simulink model "USV_Battery_MPC_First_Evaluation"  (R2025b)
settings: Solver=ode45  StartTime=0.0  StopTime=1100  MaxStep=0.1  RelTol=1e-3
model workspace (MAT data in the model file):
  battery_aware_enable = 1
  controller_mode = 2
  initial_soc = 80
  params.usv.m = 120
  params.usv.Cd = 25
  params.usv.T_max = 200
  params.usv.T_min = 0
  params.usv.u_max = 3.5
  params.usv.u_init = 0
  params.usv.x_init = 0
  params.mission.x_start = 0
  params.mission.x_dest = 1000
  params.mission.arrival_tol = 5
  params.mission.T_sim = 1100
  params.mission.dt = 0.1
  params.battery.capacity_J = 150000
  params.battery.P_aux = 10
  params.battery.initial_soc = 80
  params.battery_aware.soc_threshold_high = 60
  params.battery_aware.speed_high = 2
  params.battery_aware.soc_threshold_low = 30
  params.battery_aware.speed_med = 1.5
  params.battery_aware.speed_low = 1
  params.pid.Kp = 120
  params.pid.Ki = 15
  params.pid.Kd = 18
  params.pid.N = 50
  params.pid.anti_windup = 1
  params.mpc.Ts = 0.5
  params.mpc.Np = 15
  params.mpc.Nc = 4
  params.mpc.w_speed = 100
  params.mpc.w_power = 0.04
  params.mpc.w_rate = 0.02
  params.feasibility.min_speed_eval = 0.1
values from neighbouring files (symbols this model uses):
  waypoints = [0  0; 438.117647059  23.5294117647; 784  47.0588235294; 980  100]    [Boat_Project_Results.mat]    (also in convert_path.m = [x_waypoints, y_waypoints]; theta_waypoints.mat)
settings Model: Creator=kiran  LastModifiedBy=Ganesh

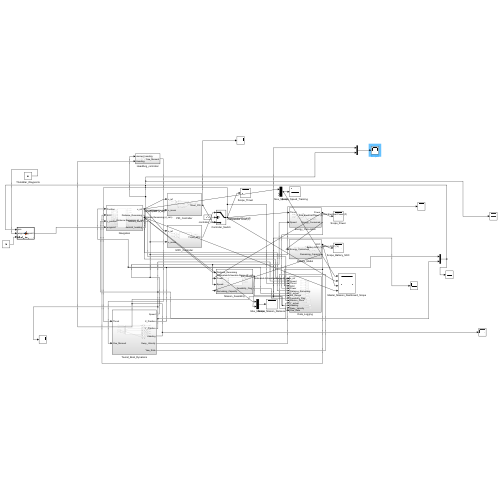
[thumbnail: Simulink's stored preview of the top-level diagram]
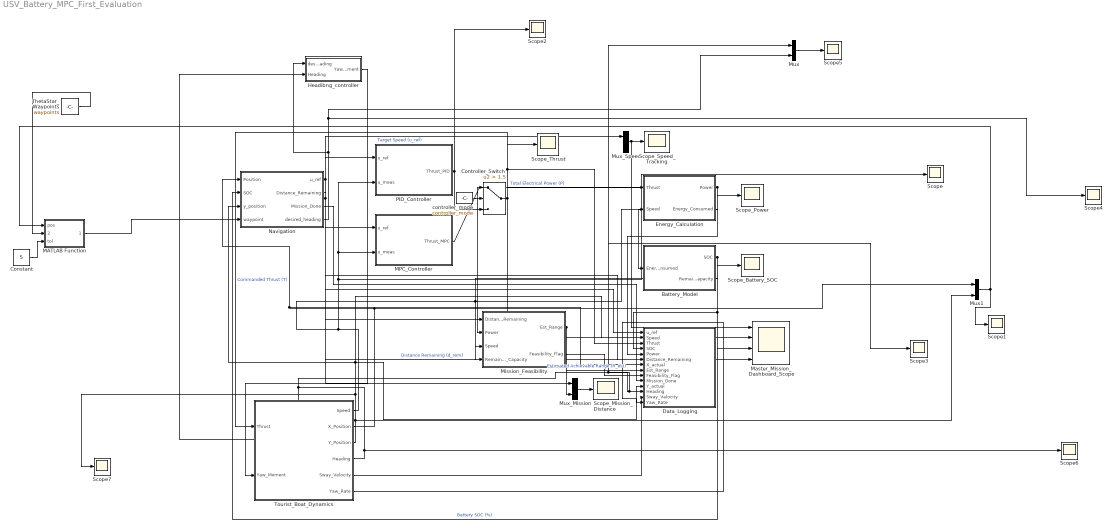
== system USV_Battery_MPC_First_Evaluation ==
  Battery_Model : Subsystem
  Constant : Constant  Value=5
  Controller_Switch : Switch  Criteria=u2 > Threshold  Threshold=1.5  SaturateOnIntegerOverflow=off  InputSameDT=off
  Data_Logging : Subsystem
  Energy_Calculation : Subsystem
  Headibng_controller : Subsystem
  MATLAB Function : MATLAB Function  TreatAsAtomicUnit=on  SystemSampleTime=0.5
  MPC_Controller : Subsystem
  Master_Mission_Dashboard_Scope : Scope  NumInputPorts=4
      settings: ActiveDisplayString=4  Title=Channel 4: Distance Remaining to Destination  ActiveDisplayYMinimum=0  ActiveDisplayYMaximum=1100  YLabel=Distance [m]
  Mission_Feasibility : Subsystem
  Mux : Mux  Inputs=2
  Mux1 : Mux  Inputs=2
  Mux_Mission : Mux  Inputs=2
  Mux_Speed : Mux  Inputs=2
  Navigation : Subsystem
  PID_Controller : Subsystem
  Scope{,1..7} (8 alike) : Scope
      Scope settings: ActiveDisplayYMinimum=-1  ActiveDisplayYMaximum=1
      Scope1 settings: ActiveDisplayYMinimum=-351.05516917665  ActiveDisplayYMaximum=1380.5211425113021  DataLoggingVariableName=ScopeData2
      Scope2 settings: ActiveDisplayYMinimum=-24.999999999999993  ActiveDisplayYMaximum=225  DataLoggingVariableName=ScopeData3
      Scope3 settings: ActiveDisplayYMinimum=-1  ActiveDisplayYMaximum=1  DataLoggingVariableName=ScopeData4
      Scope4 settings: ActiveDisplayYMinimum=-1  ActiveDisplayYMaximum=1  DataLoggingVariableName=ScopeData5
      Scope5 settings: ActiveDisplayYMinimum=-1.3769373478351028  ActiveDisplayYMaximum=4.4168787257964723  DataLoggingVariableName=ScopeData6
      Scope6 settings: ActiveDisplayYMinimum=-1  ActiveDisplayYMaximum=1  DataLoggingVariableName=ScopeData8
      Scope7 settings: DataLoggingVariableName=ScopeData10
  Scope_Battery_SOC : Scope
      settings: Title=Battery State of Charge (SOC)  ActiveDisplayYMinimum=0  ActiveDisplayYMaximum=100  YLabel=SOC [%]
  Scope_Mission_Distance : Scope
      settings: Title=Mission Navigation: Distance Remaining vs Estimated Range  ActiveDisplayYMinimum=-3805.3829127727518  ActiveDisplayYMaximum=7129.0337407343386  YLabel=Distance [meters]
  Scope_Power : Scope
      settings: Title=Instantaneous Electrical Power Draw  ActiveDisplayYMinimum=0  ActiveDisplayYMaximum=250  YLabel=Power [Watts]
  Scope_Speed_Tracking : Scope
      settings: Title=USV Speed Tracking: Target vs Measured Speed  ActiveDisplayYMinimum=0  ActiveDisplayYMaximum=2.5  YLabel=Speed [m/s]
  Scope_Thrust : Scope
      settings: Title=USV Propeller Thrust Command  ActiveDisplayYMinimum=0  ActiveDisplayYMaximum=210  YLabel=Thrust Force [N]
  ThetaStar_Waypoints : Constant  Value=waypoints
  Tourist_Boat_Dynamics : Subsystem
  controller_mode : Constant  Value=controller_mode  VectorParams1D=off
  wires:
  Battery_Model/1(SOC) -> Navigation/2(SOC), Data_Logging/4(SOC), Scope_Battery_SOC/1, Master_Mission_Dashboard_Scope/3  "Battery SOC (%)"
  Navigation/1(u_ref) -> Data_Logging/1(u_ref), PID_Controller/1(u_ref), MPC_Controller/1(u_ref), Mux_Speed/1  "Target Speed (u_ref)"
  MPC_Controller/1(Thrust_MPC) -> Controller_Switch/1
  controller_mode/1 -> Controller_Switch/2
  PID_Controller/1(Thrust_PID) -> Scope2/1, Controller_Switch/3
  Controller_Switch/1 -> Tourist_Boat_Dynamics/1(Thrust), Data_Logging/3(Thrust), Energy_Calculation/1(Thrust), Scope_Thrust/1, Master_Mission_Dashboard_Scope/2  "Commanded Thrust (T)"
  Energy_Calculation/2(Energy_Consumed) -> Battery_Model/1(Energy_Consumed)
  Navigation/2(Distance_Remaining) -> Data_Logging/6(Distance_Remaining), Mission_Feasibility/1(Distance_Remaining), Mux_Mission/1, Master_Mission_Dashboard_Scope/4  "Distance Remaining (d_rem)"
  Energy_Calculation/1(Power) -> Mission_Feasibility/2(Power), Data_Logging/5(Power), Scope_Power/1  "Total Electrical Power (P)"
  Battery_Model/2(Remaining_Capacity) -> Mission_Feasibility/4(Remaining_Capacity)
  Mission_Feasibility/1(Est_Range) -> Data_Logging/8(Est_Range), Mux_Mission/2  "Estimated Achievable Range (R_est)"
  Mission_Feasibility/2(Feasibility_Flag) -> Data_Logging/9(Feasibility_Flag)
  Mux_Speed/1 -> Scope_Speed_Tracking/1, Master_Mission_Dashboard_Scope/1
  Mux_Mission/1 -> Scope_Mission_Distance/1
  Navigation/3(Mission_Done) -> Data_Logging/10(Mission_Done)
  Tourist_Boat_Dynamics/1(Speed) -> Mission_Feasibility/3(Speed), Energy_Calculation/2(Speed), MPC_Controller/2(u_meas), PID_Controller/2(u_meas), Scope/1
  Tourist_Boat_Dynamics/2(X_Position) -> Mux1/1, Data_Logging/7(X_actual), Navigation/1(Position)
  Tourist_Boat_Dynamics/3(Y_Position) -> Scope7/1, Navigation/3(y_position), Data_Logging/11(Y_actual), Data_Logging/2(Speed), Mux1/2
  Tourist_Boat_Dynamics/4(Heading) -> Scope6/1, Data_Logging/12(Heading), Scope3/1, Mux/1, Headibng_controller/2(Heading)
  Tourist_Boat_Dynamics/5(Sway_Velocity) -> Data_Logging/13(Sway_Velocity)
  Tourist_Boat_Dynamics/6(Yaw_Rate) -> Data_Logging/14(Yaw_Rate)
  Navigation/4(desired_heading) -> Scope4/1, Mux/2, Headibng_controller/1(desired_heading)
  Mux/1 -> Scope5/1
  Headibng_controller/1(Yaw_Moment) -> Tourist_Boat_Dynamics/2(Yaw_Moment)
  ThetaStar_Waypoints/1 -> MATLAB Function/2(waypoints)
  Constant/1 -> MATLAB Function/3(tol)
  Mux1/1 -> Scope1/1, MATLAB Function/1(pos)
  MATLAB Function/1(waypoint) -> Navigation/4(waypoint)

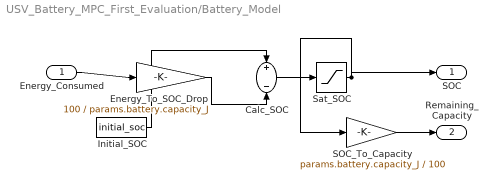
== system USV_Battery_MPC_First_Evaluation/Battery_Model ==
  Energy_Consumed : Inport
  Calc_SOC : Sum  Inputs=+-
  Energy_To_SOC_Drop : Gain  Gain=100 / params.battery.capacity_J
  Initial_SOC : Constant  Value=initial_soc
  SOC_To_Capacity : Gain  Gain=params.battery.capacity_J / 100
  Sat_SOC : Saturate  UpperLimit=100.0  LowerLimit=0.0
  SOC : Outport
  Remaining_Capacity : Outport  Port=2
  wires:
  Energy_Consumed/1 -> Energy_To_SOC_Drop/1
  Initial_SOC/1 -> Calc_SOC/1
  Energy_To_SOC_Drop/1 -> Calc_SOC/2
  Calc_SOC/1 -> Sat_SOC/1
  Sat_SOC/1 -> SOC/1, SOC_To_Capacity/1
  SOC_To_Capacity/1 -> Remaining_Capacity/1

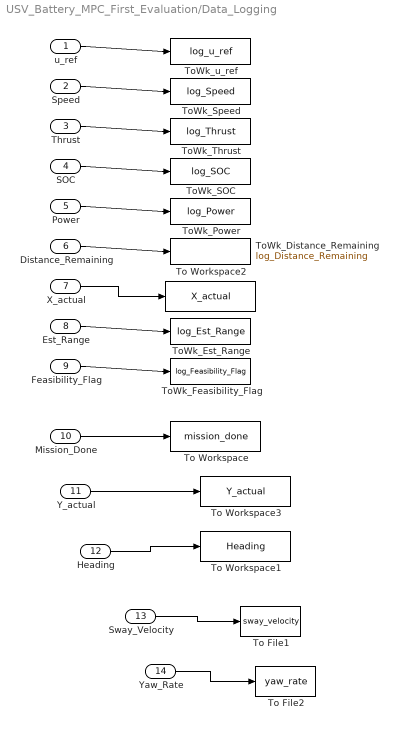
== system USV_Battery_MPC_First_Evaluation/Data_Logging ==
  u_ref : Inport
  Speed : Inport  Port=2
  Thrust : Inport  Port=3
  SOC : Inport  Port=4
  Power : Inport  Port=5
  Distance_Remaining : Inport  Port=6
  X_actual : Inport  Port=7
  Est_Range : Inport  Port=8
  Feasibility_Flag : Inport  Port=9
  Mission_Done : Inport  Port=10
  Y_actual : Inport  Port=11
  Heading : Inport  Port=12
  Sway_Velocity : Inport  Port=13
  Yaw_Rate : Inport  Port=14
  To File1 : ToFile  Filename=sway_velocity  SaveFormat=Timeseries
  To File2 : ToFile  Filename=yaw_rate  SaveFormat=Timeseries
  To Workspace : ToWorkspace  VariableName=mission_done  SaveFormat=Timeseries  SampleTime=-1
  To Workspace1 : ToWorkspace  VariableName=Heading  SaveFormat=Timeseries  SampleTime=-1
  To Workspace2 : ToWorkspace  VariableName=X_actual  SaveFormat=Timeseries  SampleTime=-1
  To Workspace3 : ToWorkspace  VariableName=Y_actual  SaveFormat=Timeseries  SampleTime=-1
  ToWk_Distance_Remaining : ToWorkspace  VariableName=log_Distance_Remaining  SaveFormat=Timeseries  SampleTime=-1
  ToWk_Est_Range : ToWorkspace  VariableName=log_Est_Range  SaveFormat=Timeseries  SampleTime=-1
  ToWk_Feasibility_Flag : ToWorkspace  VariableName=log_Feasibility_Flag  SaveFormat=Timeseries  SampleTime=-1
  ToWk_Power : ToWorkspace  VariableName=log_Power  SaveFormat=Timeseries  SampleTime=-1
  ToWk_SOC : ToWorkspace  VariableName=log_SOC  SaveFormat=Timeseries  SampleTime=-1
  ToWk_Speed : ToWorkspace  VariableName=log_Speed  SaveFormat=Timeseries  SampleTime=-1
  ToWk_Thrust : ToWorkspace  VariableName=log_Thrust  SaveFormat=Timeseries  SampleTime=-1
  ToWk_u_ref : ToWorkspace  VariableName=log_u_ref  SaveFormat=Timeseries  SampleTime=-1
  wires:
  u_ref/1 -> ToWk_u_ref/1
  Speed/1 -> ToWk_Speed/1
  Thrust/1 -> ToWk_Thrust/1
  SOC/1 -> ToWk_SOC/1
  Power/1 -> ToWk_Power/1
  Distance_Remaining/1 -> ToWk_Distance_Remaining/1
  Est_Range/1 -> ToWk_Est_Range/1
  Feasibility_Flag/1 -> ToWk_Feasibility_Flag/1
  Mission_Done/1 -> To Workspace/1
  Y_actual/1 -> To Workspace3/1
  Heading/1 -> To Workspace1/1
  Sway_Velocity/1 -> To File1/1
  Yaw_Rate/1 -> To File2/1
  X_actual/1 -> To Workspace2/1

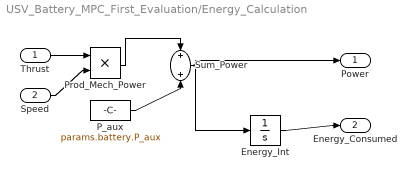
== system USV_Battery_MPC_First_Evaluation/Energy_Calculation ==
  Thrust : Inport
  Speed : Inport  Port=2
  Energy_Int : Integrator  InitialCondition=0.0
  P_aux : Constant  Value=params.battery.P_aux
  Prod_Mech_Power : Product
  Sum_Power : Sum
  Power : Outport
  Energy_Consumed : Outport  Port=2
  wires:
  Thrust/1 -> Prod_Mech_Power/1
  Speed/1 -> Prod_Mech_Power/2
  Prod_Mech_Power/1 -> Sum_Power/1
  P_aux/1 -> Sum_Power/2
  Sum_Power/1 -> Power/1, Energy_Int/1
  Energy_Int/1 -> Energy_Consumed/1

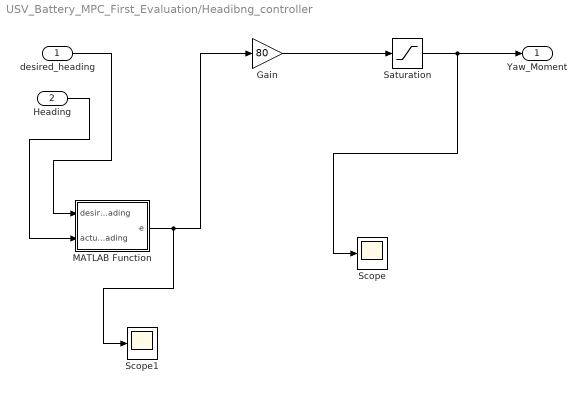
== system USV_Battery_MPC_First_Evaluation/Headibng_controller ==
  desired_heading : Inport
  Heading : Inport  Port=2
  Gain : Gain  Gain=80
  MATLAB Function : MATLAB Function  TreatAsAtomicUnit=on
  Saturation : Saturate  UpperLimit=50  LowerLimit=-50
  Scope : Scope
      settings: ActiveDisplayYMinimum=-1  ActiveDisplayYMaximum=1  DataLoggingVariableName=ScopeData7
  Scope1 : Scope
      settings: ActiveDisplayYMinimum=-1  ActiveDisplayYMaximum=1  DataLoggingVariableName=ScopeData9
  Yaw_Moment : Outport
  wires:
  desired_heading/1 -> MATLAB Function/1(desired_heading)
  Heading/1 -> MATLAB Function/2(actual_heading)
  Saturation/1 -> Scope/1, Yaw_Moment/1
  Gain/1 -> Saturation/1
  MATLAB Function/1(e) -> Scope1/1, Gain/1

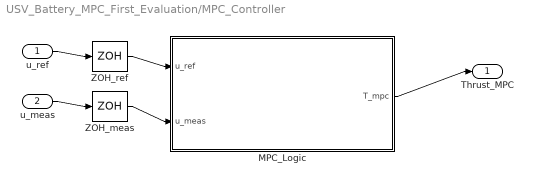
== system USV_Battery_MPC_First_Evaluation/MPC_Controller ==
  u_ref : Inport
  u_meas : Inport  Port=2
  MPC_Logic : MATLAB Function  TreatAsAtomicUnit=on
  ZOH_meas : ZeroOrderHold  SampleTime=params.mpc.Ts
  ZOH_ref : ZeroOrderHold  SampleTime=params.mpc.Ts
  Thrust_MPC : Outport
  wires:
  u_ref/1 -> ZOH_ref/1
  u_meas/1 -> ZOH_meas/1
  ZOH_ref/1 -> MPC_Logic/1(u_ref)
  ZOH_meas/1 -> MPC_Logic/2(u_meas)
  MPC_Logic/1(T_mpc) -> Thrust_MPC/1

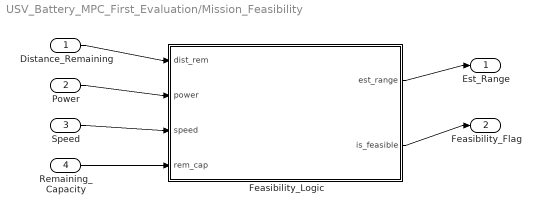
== system USV_Battery_MPC_First_Evaluation/Mission_Feasibility ==
  Distance_Remaining : Inport
  Power : Inport  Port=2
  Speed : Inport  Port=3
  Remaining_Capacity : Inport  Port=4
  Feasibility_Logic : MATLAB Function  TreatAsAtomicUnit=on
  Est_Range : Outport
  Feasibility_Flag : Outport  Port=2
  wires:
  Distance_Remaining/1 -> Feasibility_Logic/1(dist_rem)
  Power/1 -> Feasibility_Logic/2(power)
  Speed/1 -> Feasibility_Logic/3(speed)
  Remaining_Capacity/1 -> Feasibility_Logic/4(rem_cap)
  Feasibility_Logic/1(est_range) -> Est_Range/1
  Feasibility_Logic/2(is_feasible) -> Feasibility_Flag/1

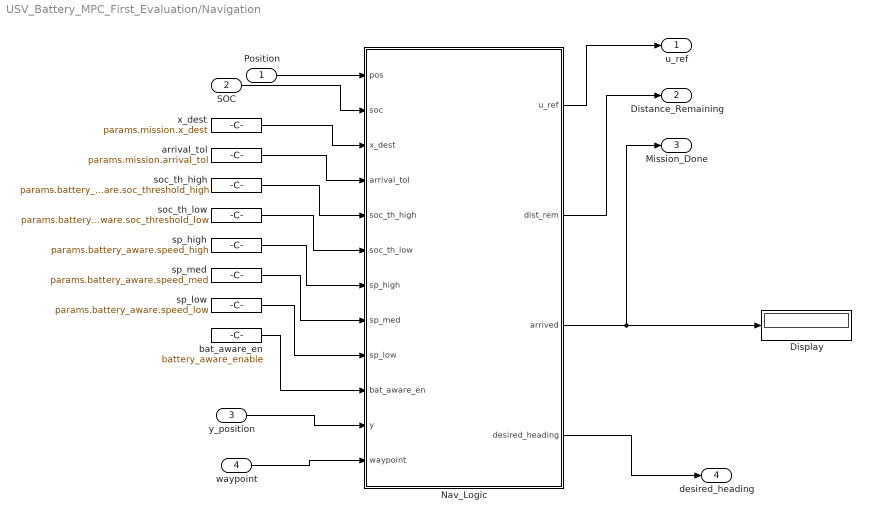
== system USV_Battery_MPC_First_Evaluation/Navigation ==
  Position : Inport
  SOC : Inport  Port=2
  y_position : Inport  Port=3
  waypoint : Inport  Port=4
  Display : Display
  Nav_Logic : MATLAB Function  TreatAsAtomicUnit=on
  arrival_tol : Constant  Value=params.mission.arrival_tol
  bat_aware_en : Constant  Value=battery_aware_enable
  soc_th_high : Constant  Value=params.battery_aware.soc_threshold_high
  soc_th_low : Constant  Value=params.battery_aware.soc_threshold_low
  sp_high : Constant  Value=params.battery_aware.speed_high
  sp_low : Constant  Value=params.battery_aware.speed_low
  sp_med : Constant  Value=params.battery_aware.speed_med
  x_dest : Constant  Value=params.mission.x_dest
  u_ref : Outport
  Distance_Remaining : Outport  Port=2
  Mission_Done : Outport  Port=3
  desired_heading : Outport  Port=4
  wires:
  Position/1 -> Nav_Logic/1(pos)
  SOC/1 -> Nav_Logic/2(soc)
  x_dest/1 -> Nav_Logic/3(x_dest)
  arrival_tol/1 -> Nav_Logic/4(arrival_tol)
  soc_th_high/1 -> Nav_Logic/5(soc_th_high)
  soc_th_low/1 -> Nav_Logic/6(soc_th_low)
  sp_high/1 -> Nav_Logic/7(sp_high)
  sp_med/1 -> Nav_Logic/8(sp_med)
  sp_low/1 -> Nav_Logic/9(sp_low)
  bat_aware_en/1 -> Nav_Logic/10(bat_aware_en)
  Nav_Logic/1(u_ref) -> u_ref/1
  Nav_Logic/2(dist_rem) -> Distance_Remaining/1
  Nav_Logic/3(arrived) -> Display/1, Mission_Done/1
  y_position/1 -> Nav_Logic/11(y)
  Nav_Logic/4(desired_heading) -> desired_heading/1
  waypoint/1 -> Nav_Logic/12(waypoint)

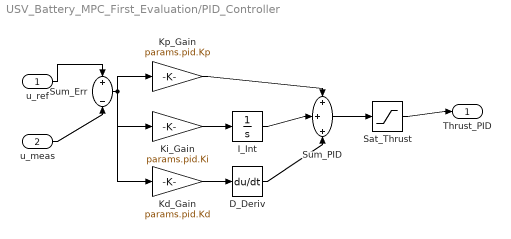
== system USV_Battery_MPC_First_Evaluation/PID_Controller ==
  u_ref : Inport
  u_meas : Inport  Port=2
  D_Deriv : Derivative
  I_Int : Integrator  LimitOutput=on  UpperSaturationLimit=params.usv.T_max  LowerSaturationLimit=params.usv.T_min
  Kd_Gain : Gain  Gain=params.pid.Kd
  Ki_Gain : Gain  Gain=params.pid.Ki
  Kp_Gain : Gain  Gain=params.pid.Kp
  Sat_Thrust : Saturate  UpperLimit=params.usv.T_max  LowerLimit=params.usv.T_min
  Sum_Err : Sum  Inputs=+-
  Sum_PID : Sum  Inputs=+++
  Thrust_PID : Outport
  wires:
  u_ref/1 -> Sum_Err/1
  u_meas/1 -> Sum_Err/2
  Sum_Err/1 -> Kp_Gain/1, Ki_Gain/1, Kd_Gain/1
  Ki_Gain/1 -> I_Int/1
  Kd_Gain/1 -> D_Deriv/1
  Kp_Gain/1 -> Sum_PID/1
  I_Int/1 -> Sum_PID/2
  D_Deriv/1 -> Sum_PID/3
  Sum_PID/1 -> Sat_Thrust/1
  Sat_Thrust/1 -> Thrust_PID/1

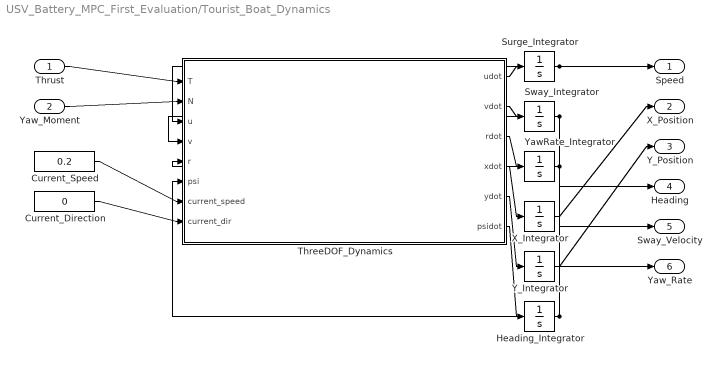
== system USV_Battery_MPC_First_Evaluation/Tourist_Boat_Dynamics ==
  Thrust : Inport
  Yaw_Moment : Inport  Port=2
  Current_Direction : Constant  Value=0
  Current_Speed : Constant  Value=0.2
  Heading_Integrator : Integrator
  Surge_Integrator : Integrator  LimitOutput=on  UpperSaturationLimit=params.usv.u_max  LowerSaturationLimit=0.0
  Sway_Integrator : Integrator
  ThreeDOF_Dynamics : MATLAB Function  TreatAsAtomicUnit=on
  X_Integrator : Integrator
  Y_Integrator : Integrator
  YawRate_Integrator : Integrator
  Speed : Outport
  X_Position : Outport  Port=2
  Y_Position : Outport  Port=3
  Heading : Outport  Port=4
  Sway_Velocity : Outport  Port=5
  Yaw_Rate : Outport  Port=6
  wires:
  Thrust/1 -> ThreeDOF_Dynamics/1(T)
  Yaw_Moment/1 -> ThreeDOF_Dynamics/2(N)
  Surge_Integrator/1 -> ThreeDOF_Dynamics/3(u), Speed/1
  Sway_Integrator/1 -> ThreeDOF_Dynamics/4(v), Sway_Velocity/1
  YawRate_Integrator/1 -> ThreeDOF_Dynamics/5(r), Yaw_Rate/1
  Heading_Integrator/1 -> ThreeDOF_Dynamics/6(psi), Heading/1
  Current_Speed/1 -> ThreeDOF_Dynamics/7(current_speed)
  Current_Direction/1 -> ThreeDOF_Dynamics/8(current_dir)
  ThreeDOF_Dynamics/1(udot) -> Surge_Integrator/1
  ThreeDOF_Dynamics/2(vdot) -> Sway_Integrator/1
  ThreeDOF_Dynamics/3(rdot) -> YawRate_Integrator/1
  ThreeDOF_Dynamics/4(xdot) -> X_Integrator/1
  ThreeDOF_Dynamics/5(ydot) -> Y_Integrator/1
  ThreeDOF_Dynamics/6(psidot) -> Heading_Integrator/1
  X_Integrator/1 -> X_Position/1
  Y_Integrator/1 -> Y_Position/1

== matlab function USV_Battery_MPC_First_Evaluation/MPC_Controller/MPC_Logic ==
  data: u_ref input size=1; T_mpc output size=1; u_meas input size=1
function T_mpc = MPC_Logic(u_ref, u_meas)
coder.extrinsic('mpc_controller', 'parameters');
T_mpc = 0.0;
persistent T_prev;
if isempty(T_prev)
    T_prev = 0.0;
end
p = parameters();
T_opt = 0.0;
T_opt = mpc_controller(u_meas, u_ref, T_prev, p);
T_mpc = double(T_opt);
T_prev = T_mpc;
end

== matlab function USV_Battery_MPC_First_Evaluation/Navigation/Nav_Logic ==
  data: pos input size=1; u_ref output size=1; soc input size=1; x_dest input size=1; arrival_tol input size=1; soc_th_high input size=1; soc_th_low input size=1; sp_high input size=1; sp_med input size=1; sp_low input size=1; bat_aware_en input size=1; y input; waypoint input; dist_rem output size=1; arrived output size=1; desired_heading output

function [u_ref, dist_rem, arrived, desired_heading] = ...
    Nav_Logic(pos, soc, x_dest, arrival_tol, ...
    soc_th_high, soc_th_low, sp_high, sp_med, ...
    sp_low, bat_aware_en, y, waypoint)

% Initialize outputs
u_ref = 0.0;
arrived = 0.0;
desired_heading = 0.0;

% Read selected waypoint
x_dest = waypoint(1);
y_dest = waypoint(2);

% Calculate 2D distance
dx = x_dest - pos;
dy = y_dest - y;
dist_rem = sqrt(dx^2 + dy^2);

% Calculate desired heading
desired_heading = atan2(dy, dx);

% Check arrival
if dist_rem <= arrival_tol
    u_ref = 0.0;
    arrived = 1.0;
else
    arrived = 0.0;

    % Battery-aware speed selection
    if bat_aware_en > 0.5
        if soc > soc_th_high
            u_ref = sp_high;
        elseif soc >= soc_th_low
            u_ref = sp_med;
        else
            u_ref = sp_low;
        end
    else
        u_ref = sp_high;
    end
end

end

== matlab function USV_Battery_MPC_First_Evaluation/Mission_Feasibility/Feasibility_Logic ==
  data: dist_rem input size=1; est_range output size=1; power input size=1; speed input size=1; rem_cap input size=1; is_feasible output size=1
function [est_range, is_feasible] = Feasibility_Logic(dist_rem, power, speed, rem_cap)
est_range = 0.0;
is_feasible = 0.0;
eff_speed = max(speed, 0.1);
e_per_m = power / eff_speed;
est_range = rem_cap / max(e_per_m, 0.01);
if est_range >= dist_rem
    is_feasible = 1.0;
else
    is_feasible = 0.0;
end
end

== matlab function USV_Battery_MPC_First_Evaluation/Tourist_Boat_Dynamics/ThreeDOF_Dynamics ==
  data: T input size=1; N input size=1; u input size=1; udot output size=1; v input size=1; r input size=1; psi input size=1; current_speed input size=1; current_dir input size=1; vdot output size=1; rdot output size=1; xdot output size=1; ydot output size=1; psidot output size=1
function [udot, vdot, rdot, xdot, ydot, psidot] = ...
    ThreeDOF_Dynamics(T, N, u, v, r, psi, current_speed, current_dir)

% Boat parameters
m = 120.0;
Iz = 2500.0;
Cd = 25.0;
Xu = 25.0;
Yv = 50.0;
Nr = 600.0;

% River current in earth-fixed frame
uc = current_speed * cos(current_dir);
vc = current_speed * sin(current_dir);

% Convert current to body-fixed frame
u_c_body = uc * cos(psi) + vc * sin(psi);
v_c_body = -uc * sin(psi) + vc * cos(psi);

% Relative velocity with respect to water
u_rel = u - u_c_body;
v_rel = v - v_c_body;

% Hydrodynamic forces
X = T - Xu * u_rel - Cd * u_rel * abs(u_rel);
Y = -Yv * v_rel;

% Hydrodynamic yaw moment
N_hydro = -Nr * r;

% 3-DOF equations of motion
udot = (X + m * v * r) / m;
vdot = (Y - m * u * r) / m;
rdot = (N + N_hydro) / Iz;

% Earth-fixed kinematics
xdot = u * cos(psi) - v * sin(psi);
ydot = u * sin(psi) + v * cos(psi);
psidot = r;

end

== matlab function USV_Battery_MPC_First_Evaluation/Headibng_controller/MATLAB Function ==
  data: desired_heading input; e output; actual_heading input
function e = heading_error(desired_heading, actual_heading)
    e = desired_heading - actual_heading;
    e = atan2(sin(e), cos(e));
end

== matlab function USV_Battery_MPC_First_Evaluation/MATLAB Function ==
  data: pos input; waypoint output; waypoints input; tol input
function waypoint = Select_Waypoint(pos, waypoints, tol)

persistent idx

if isempty(idx)
    idx = 1;
end

n = size(waypoints,1);

while idx < n
    dx = waypoints(idx,1) - pos(1);
    dy = waypoints(idx,2) - pos(2);

    if hypot(dx,dy) <= tol
        idx = idx + 1;
    else
        break;
    end
end

waypoint = waypoints(idx,:)';
end
